simulink model "QDrone_Recenter_CSV_Test"  (R2021b)
settings: Solver=FixedStepDiscrete  StartTime=0.0  StopTime=sim_stop_time  FixedStep=1/30  RelTol=1e-3
settings Model: Creator=user  LastModifiedBy=user

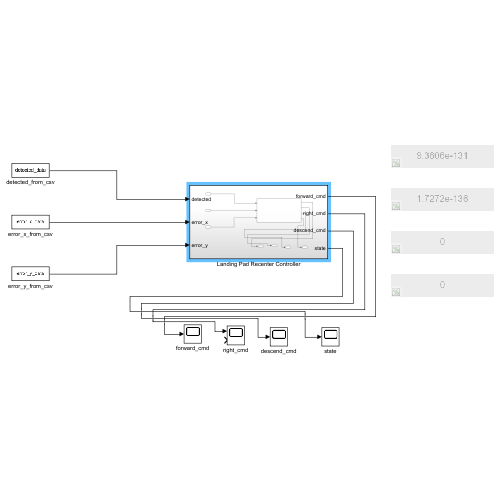
[thumbnail: Simulink's stored preview of the top-level diagram]
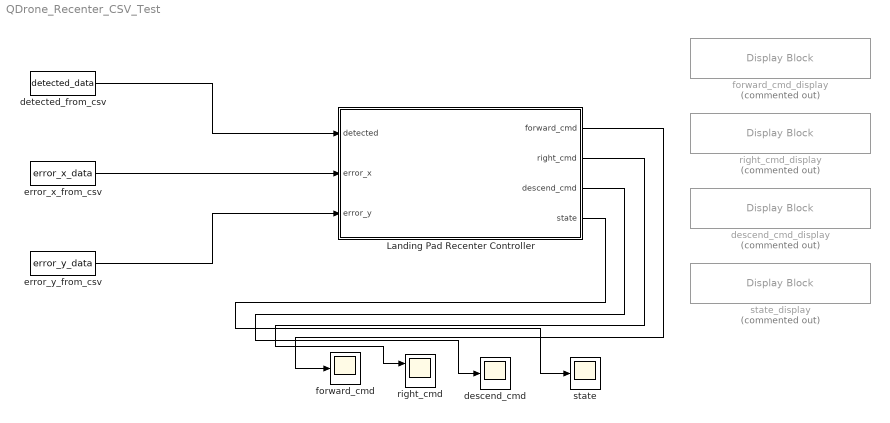
== system QDrone_Recenter_CSV_Test ==
  Landing Pad Recenter Controller : Subsystem
  descend_cmd : Scope
  descend_cmd_display : DisplayBlock  Commented=on  LabelPosition=Hide  Format=short  Transparency=1
  detected_from_csv : FromWorkspace  VariableName=detected_data
  error_x_from_csv : FromWorkspace  VariableName=error_x_data
  error_y_from_csv : FromWorkspace  VariableName=error_y_data
  forward_cmd : Scope
  forward_cmd_display : DisplayBlock  Commented=on  LabelPosition=Hide  Format=short  Transparency=1
  right_cmd : Scope  NumInputPorts=2
  "right_cmd_display " : DisplayBlock  Commented=on  LabelPosition=Hide  Format=short  Transparency=1
  state : Scope
  state_display : DisplayBlock  Commented=on  LabelPosition=Hide  Format=short  Transparency=1
  wires:
  detected_from_csv/1 -> Landing Pad Recenter Controller/1(detected)
  error_x_from_csv/1 -> Landing Pad Recenter Controller/2(error_x)
  error_y_from_csv/1 -> Landing Pad Recenter Controller/3(error_y)
  Landing Pad Recenter Controller/1(forward_cmd) -> forward_cmd/1
  Landing Pad Recenter Controller/2(right_cmd) -> right_cmd/1
  Landing Pad Recenter Controller/3(descend_cmd) -> descend_cmd/1
  Landing Pad Recenter Controller/4(state) -> state/1

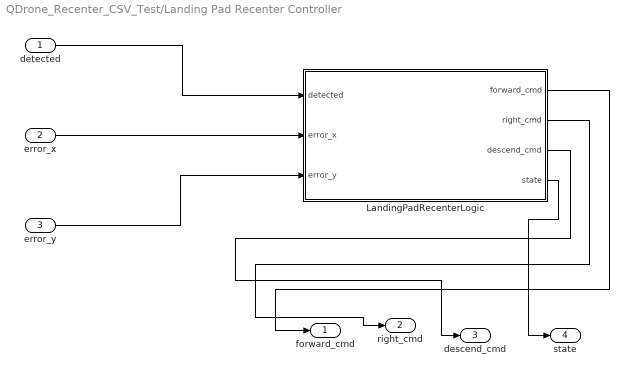
== system QDrone_Recenter_CSV_Test/Landing Pad Recenter Controller ==
  detected : Inport
  error_x : Inport  Port=2
  error_y : Inport  Port=3
  LandingPadRecenterLogic : MATLAB Function  TreatAsAtomicUnit=on
  forward_cmd : Outport
  right_cmd : Outport  Port=2
  descend_cmd : Outport  Port=3
  state : Outport  Port=4
  wires:
  error_y/1 -> LandingPadRecenterLogic/3(error_y)
  LandingPadRecenterLogic/3(descend_cmd) -> descend_cmd/1
  LandingPadRecenterLogic/2(right_cmd) -> right_cmd/1
  LandingPadRecenterLogic/1(forward_cmd) -> forward_cmd/1
  LandingPadRecenterLogic/4(state) -> state/1
  error_x/1 -> LandingPadRecenterLogic/2(error_x)
  detected/1 -> LandingPadRecenterLogic/1(detected)

== matlab function QDrone_Recenter_CSV_Test/Landing Pad Recenter Controller/LandingPadRecenterLogic ==
  data: detected input; forward_cmd output; error_x input; error_y input; right_cmd output; descend_cmd output; state output
function [forward_cmd, right_cmd, descend_cmd, state] = LandingPadRecenterLogic(detected, error_x, error_y)

% Inputs:
% detected : 1 if YOLO detects landing pad, 0 otherwise
% error_x  : pad_center_x - image_center_x
% error_y  : pad_center_y - image_center_y

% Outputs:
% forward_cmd : positive = move forward, negative = move backward
% right_cmd   : positive = move right, negative = move left
% descend_cmd : positive small descent command when landing is ready
% state       : 0 no detection, 1 recentering, 2 centered, 3 landing ready

persistent smooth_forward smooth_right centered_counter

if isempty(smooth_forward)
    smooth_forward = 0;
    smooth_right = 0;
    centered_counter = 0;
end

% Tunable parameters
deadband_pixels = 40;
alpha = 0.25;
max_cmd = 0.20;          
centered_required = 10;
descend_speed = 0.05;

raw_forward = 0;
raw_right = 0;
descend_cmd = 0;
state = 0;

% Your image size is 640x480
image_center_x = 320;
image_center_y = 240;

if detected == 1

    x_centered = abs(error_x) <= deadband_pixels;
    y_centered = abs(error_y) <= deadband_pixels;

    if x_centered && y_centered
        centered_counter = centered_counter + 1;
        state = 2;
    else
        centered_counter = 0;
        state = 1;

        % Calibration-confirmed mapping:
        % error_x > 0 -> move backward
        % error_x < 0 -> move forward
        if ~x_centered
            raw_forward = -error_x / image_center_x;
        end

        % error_y > 0 -> move left
        % error_y < 0 -> move right
        if ~y_centered
            raw_right = -error_y / image_center_y;
        end

        raw_forward = min(max(raw_forward, -1), 1);
        raw_right = min(max(raw_right, -1), 1);
    end

    if centered_counter >= centered_required
        state = 3;
        descend_cmd = descend_speed;
        raw_forward = 0;
        raw_right = 0;
    end

else
    centered_counter = 0;
    state = 0;
    raw_forward = 0;
    raw_right = 0;
end

% Smooth commands
smooth_forward = alpha * raw_forward + (1 - alpha) * smooth_forward;
smooth_right = alpha * raw_right + (1 - alpha) * smooth_right;

% Decay commands when no detection
if detected == 0
    smooth_forward = 0.7 * smooth_forward;
    smooth_right = 0.7 * smooth_right;
end

% Scale to small safe command range
forward_cmd = max_cmd * smooth_forward;
right_cmd = max_cmd * smooth_right;

end
